simulink model "chaine_qpsk"  (R2023b)
settings: Solver=FixedStepDiscrete  StartTime=0.0  StopTime=Tsim  RelTol=1e-3
values from neighbouring files (symbols this model uses):
  graine = 1    [extension_source_huffman.m]    (also in mes_parametres.m = mod(sum(c .* (1:numel(c)) * 31) + 7 * numel(c), 2^31 - 1); parametres_chaine.m = P.graine; parametres_perso.m = mod(sum(c .* (1:numel(c)) * 31) + 7 * numel(c), 2^31 - 1); partie4_q10.m = P.graine)
  p1 = P.p1    [parametres.m]    (also in parametres_chaine.m = 0.5; partie3_q4.m; partie3_q5.m; partie3_q8.m = 0.3)
  sigma2v = N0 / 2    (= 0.0995267926384)    [partie5_q2.m]    (also in partie5_q3.m = N0 / 2; partie5_q4.m = N0 / 2; partie5_q5.m = Eb / e / 2)
  tabB1 = [0 0 1 1]    [partie5_q2.m]    (also in partie5_q3.m; partie5_q4.m; partie5_q5.m = M(m).tabB1)
  tabB2 = [0 1 0 1]    [partie5_q2.m]    (also in partie5_q3.m; partie5_q4.m; partie5_q5.m = M(m).tabB2)
  tabI = [ 1  1 -1 -1] / sqrt(2)    [partie5_q2.m]    (also in partie5_q3.m = [1 1 -1 -1] / sqrt(2); partie5_q4.m = [1 1 -1 -1] / sqrt(2); partie5_q5.m = M(m).tabI)
  tabQ = [ 1 -1  1 -1] / sqrt(2)    [partie5_q2.m]    (also in partie5_q3.m = [1 -1 1 -1] / sqrt(2); partie5_q4.m = [1 -1 1 -1] / sqrt(2); partie5_q5.m = M(m).tabQ)
  Tb = 1    [parametres.m]    (also in parametres_chaine.m; partie3_simulation.m; partie4_q10.m = 7; partie5_q2.m)
  Ts = 2 * Tb    (= 2)    [partie5_q2.m]    (also in partie5_q3.m; partie5_q4.m; partie5_q5.m)
libraries: simulink x5
settings Model: Creator=e2604176  LastModifiedBy=e2604176
settings OptimizationCC: BooleanDataType=off

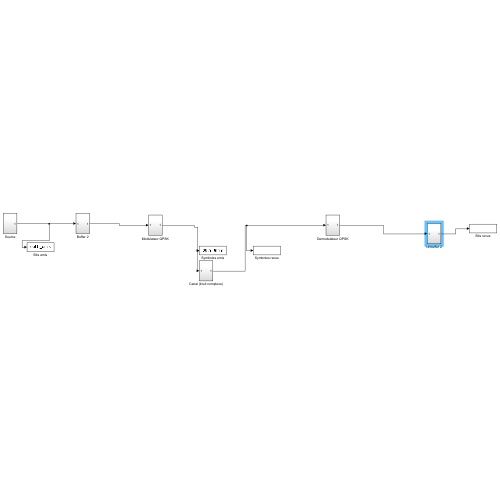
[thumbnail: Simulink's stored preview of the top-level diagram]
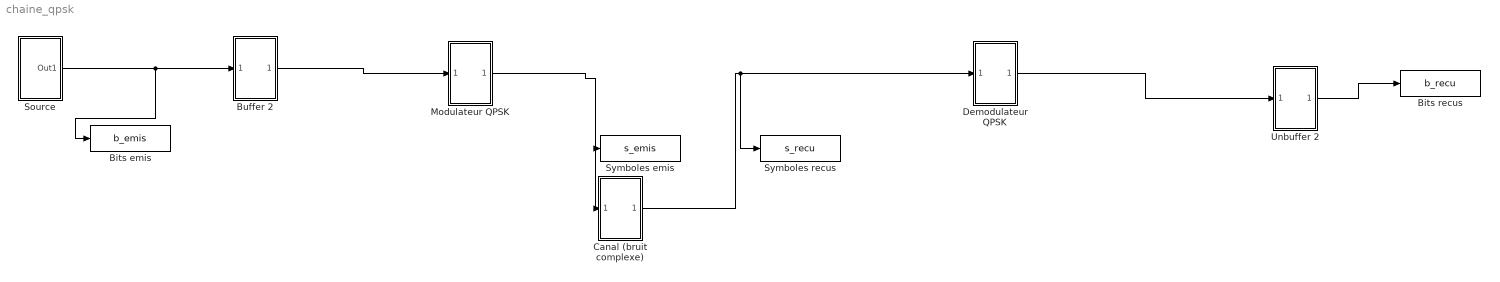
== system chaine_qpsk ==
  Bits emis : ToWorkspace  VariableName=b_emis  SampleTime=-1
  Bits recus : ToWorkspace  VariableName=b_recu  SampleTime=-1
  Buffer 2 : Subsystem
  Canal (bruit complexe) : Subsystem
  Demodulateur QPSK : Subsystem
  Modulateur QPSK : Subsystem
  Source : Subsystem
  Symboles emis : ToWorkspace  VariableName=s_emis  SampleTime=-1
  Symboles recus : ToWorkspace  VariableName=s_recu  SampleTime=-1
  Unbuffer 2 : Subsystem
  wires:
  Source/1(Out1) -> Buffer 2/1(In1), Bits emis/1
  Modulateur QPSK/1(Out1) -> Canal (bruit complexe)/1(In1), Symboles emis/1
  Buffer 2/1(Out1) -> Modulateur QPSK/1(In1)
  Canal (bruit complexe)/1(Out1) -> Symboles recus/1, Demodulateur QPSK/1(In1)
  Demodulateur QPSK/1(Out1) -> Unbuffer 2/1(In1)
  Unbuffer 2/1(Out1) -> Bits recus/1

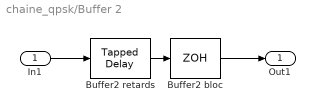
== system chaine_qpsk/Buffer 2 ==
  In1 : Inport
  Buffer2 bloc : ZeroOrderHold  SampleTime=Ts
  Buffer2 retards : simulink/Discrete/Tapped Delay  vinit=0  samptime=Tb  NumDelays=1  DelayOrder=Oldest  includeCurrent=on
  Out1 : Outport
  wires:
  Buffer2 bloc/1 -> Out1/1
  Buffer2 retards/1 -> Buffer2 bloc/1
  In1/1 -> Buffer2 retards/1

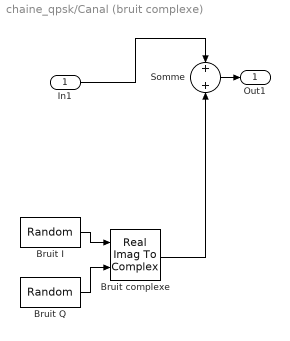
== system chaine_qpsk/Canal (bruit complexe) ==
  In1 : Inport
  Bruit I : RandomNumber  Variance=sigma2v  Seed=graine + 1  SampleTime=Ts
  Bruit Q : RandomNumber  Variance=sigma2v  Seed=graine + 2  SampleTime=Ts
  Bruit complexe : RealImagToComplex
  Somme : Sum
  Out1 : Outport
  wires:
  Bruit I/1 -> Bruit complexe/1
  Bruit Q/1 -> Bruit complexe/2
  Bruit complexe/1 -> Somme/2
  In1/1 -> Somme/1
  Somme/1 -> Out1/1

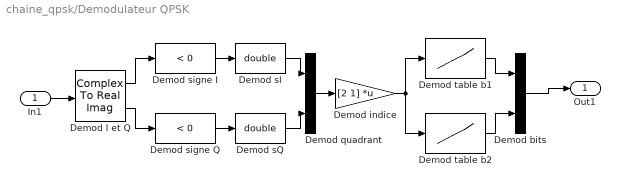
== system chaine_qpsk/Demodulateur QPSK ==
  In1 : Inport
  Demod I et Q : ComplexToRealImag
  Demod bits : Mux  Inputs=2
  Demod indice : Gain  Gain=[2 1]  Multiplication=Matrix(K*u)
  Demod quadrant : Mux  Inputs=2
  Demod sI : DataTypeConversion  OutDataTypeStr=double  SaturateOnIntegerOverflow=off  RndMeth=Floor
  Demod sQ : DataTypeConversion  OutDataTypeStr=double  SaturateOnIntegerOverflow=off  RndMeth=Floor
  Demod signe I : simulink/Logic and Bit Operations/Compare To Constant  relop=<  const=0  OutDataTypeStr=boolean
  Demod signe Q : simulink/Logic and Bit Operations/Compare To Constant  relop=<  const=0  OutDataTypeStr=boolean
  Demod table b1 : Lookup_n-D  NumberOfTableDimensions=1  BreakpointsForDimension1=0:3  Table=tabB1  InternalRulePriority=Speed  RndMeth=Simplest
  Demod table b2 : Lookup_n-D  NumberOfTableDimensions=1  BreakpointsForDimension1=0:3  Table=tabB2  InternalRulePriority=Speed  RndMeth=Simplest
  Out1 : Outport
  wires:
  Demod indice/1 -> Demod table b1/1, Demod table b2/1
  Demod bits/1 -> Out1/1
  Demod table b1/1 -> Demod bits/1
  Demod table b2/1 -> Demod bits/2
  Demod signe Q/1 -> Demod sQ/1
  In1/1 -> Demod I et Q/1
  Demod quadrant/1 -> Demod indice/1
  Demod sQ/1 -> Demod quadrant/2
  Demod signe I/1 -> Demod sI/1
  Demod I et Q/1 -> Demod signe I/1
  Demod sI/1 -> Demod quadrant/1
  Demod I et Q/2 -> Demod signe Q/1

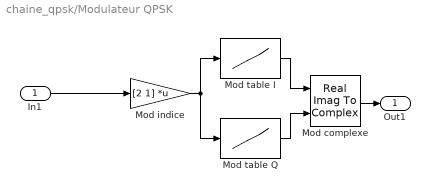
== system chaine_qpsk/Modulateur QPSK ==
  In1 : Inport
  Mod complexe : RealImagToComplex
  Mod indice : Gain  Gain=[2 1]  Multiplication=Matrix(K*u)
  Mod table I : Lookup_n-D  NumberOfTableDimensions=1  BreakpointsForDimension1=0:3  Table=tabI  InternalRulePriority=Speed  RndMeth=Simplest
  Mod table Q : Lookup_n-D  NumberOfTableDimensions=1  BreakpointsForDimension1=0:3  Table=tabQ  InternalRulePriority=Speed  RndMeth=Simplest
  Out1 : Outport
  wires:
  Mod table I/1 -> Mod complexe/1
  Mod table Q/1 -> Mod complexe/2
  In1/1 -> Mod indice/1
  Mod complexe/1 -> Out1/1
  Mod indice/1 -> Mod table I/1, Mod table Q/1

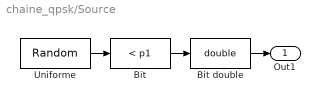
== system chaine_qpsk/Source ==
  Bit : simulink/Logic and Bit Operations/Compare To Constant  relop=<  const=p1  OutDataTypeStr=boolean
  Bit double : DataTypeConversion  OutDataTypeStr=double  SaturateOnIntegerOverflow=off  RndMeth=Floor
  Uniforme : UniformRandomNumber  Minimum=0  Seed=graine  SampleTime=Tb
  Out1 : Outport
  wires:
  Bit/1 -> Bit double/1
  Uniforme/1 -> Bit/1
  Bit double/1 -> Out1/1

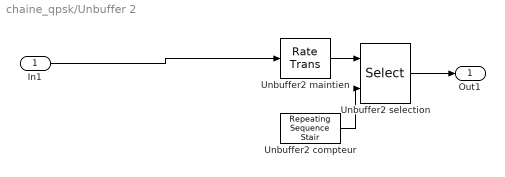
== system chaine_qpsk/Unbuffer 2 ==
  In1 : Inport
  Unbuffer2 compteur : simulink/Sources/Repeating Sequence Stair  OutValues=1:2  tsamp=Tb  OutMin=[]  OutMax=[]  OutDataTypeStr=double  OutputDataTypeScalingMode=double  OutDataType=fixdt(0,8)  ConRadixGroup=Best Precision: Vector-wise  OutScaling=2^-12
  Unbuffer2 maintien : RateTransition  OutPortSampleTime=Tb
  Unbuffer2 selection : Selector  InputPortWidth=2  IndexOptions=Index vector (port)  Indices=[1 3]  OutputSizes=1
  Out1 : Outport
  wires:
  Unbuffer2 selection/1 -> Out1/1
  Unbuffer2 maintien/1 -> Unbuffer2 selection/1
  Unbuffer2 compteur/1 -> Unbuffer2 selection/2
  In1/1 -> Unbuffer2 maintien/1
